simulink model "mcb_pmsm_nonlin_fwc"  (R2024b)
settings: Solver=FixedStepDiscrete  StartTime=0.0  StopTime=inf  RelTol=1e-3  EnableMultiTasking=on
InitFcn:
  | mcb_e11_nonlin_fwc_data;
model workspace (MAT data in the model file):
  encoderResolution = 2000
  hallOffset = '0.5'
  indexOffset = 850
  polePairs = '4'
values from neighbouring files (symbols this model uses):
  PI_params = mcb_SetControllerParameters(pmsm,inverter,PU_System,T_pwm,Ts,Ts_speed,Delays)    [mcb_pmsm_nonlin_fwc_data.m]
  pmsm =     [IPMSM_template_data.mat]    (also in mcb_pmsm_nonlin_fwc_data.m = mcbPMSMUpdateLdLqFluxPM(pmsm,PMSMLUT,round(tmpmat(1,1)),roun)
  PU_System = mcb_SetPUSystem(pmsm,inverter)    [mcb_pmsm_nonlin_fwc_data.m]
  PWM_frequency = 20e3    (= 20000)    [mcb_pmsm_nonlin_fwc_data.m]
  Ts = T_pwm    (= 5e-05)    [mcb_pmsm_nonlin_fwc_data.m]
  Ts_motor = T_pwm/2    (= 2.5e-05)    [mcb_pmsm_nonlin_fwc_data.m]
  Ts_speed = 30*Ts    (= 0.0015)    [mcb_pmsm_nonlin_fwc_data.m]
libraries: nesl_utility x11, mcbcontrolslib x9, fl_lib x8, ee_lib x7, slpidlib x3, mcbpmsmnonlinearlib x3, mcbpositiondecoderlib x2, nesl_utility_internal x2, simulink x1, eeGeneralControl x1, mcbutilslib x1
(part 2 of 2)

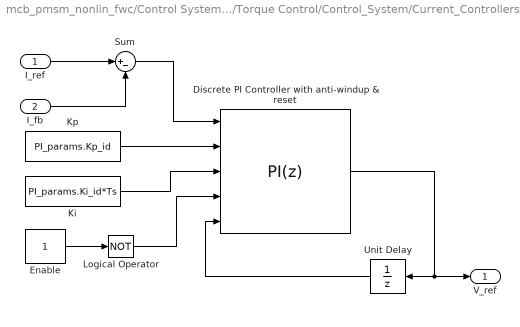
== system mcb_pmsm_nonlin_fwc/Control System/Torque Control/Control_System/Current_Controllers/PI_Controller_Id ==
  I_ref : Inport
  I_fb : Inport  Port=2
  Discrete PI Controller with anti-windup & reset : slpidlib/PID Controller  Controller=PI  Form=Parallel  TimeDomain=Discrete-time  UseExternalTs=off  SampleTime=-1  IntegratorMethod=Forward Euler  FilterMethod=Forward Euler  ControllerParametersSource=external  P=1  I=1  UseKiTs=on  D=0  UseExternalDerivativeSource=off  N=100  UseFilter=on  TunerSelectOption=Transfer Function Based (PID Tuner App)  InitialConditionSource=external  InitialConditionForIntegrator=0  InitialConditionForFilter=0  DifferentiatorICPrevScaledInput=0  ExternalReset=level  TrackingMode=off  Kt=1  LimitOutput=on  SatLimitsSource=internal  UpperSaturationLimit=1  LowerSaturationLimit=-1  LinearizeAsGain=on  AntiWindupMode=clamping  Kb=1  LimitIntegrator=off  UpperIntegratorSaturationLimit=inf  LowerIntegratorSaturationLimit=-inf  RndMeth=Simplest  POutMin=[]  POutMax=[]  IOutMin=[]  IOutMax=[]  DOutMin=[]  DOutMax=[]  NOutMin=[]  NOutMax=[]  SumOutMin=[]  SumOutMax=[]  SaturationOutDataTypeStr=Inherit: Inherit via back propagation  SaturationOutMin=[]  SaturationOutMax=[]  PParamMin=[]  PParamMax=[]  IParamMin=[]  IParamMax=[]  DParamMin=[]  DParamMax=[]  NParamMin=[]  NParamMax=[]  KbParamMin=[]  KbParamMax=[]  KtParamMin=[]  KtParamMax=[]  KbOutMin=[]  KbOutMax=[]  KtOutMin=[]  KtOutMax=[]  IntegratorOutMin=[]  IntegratorOutMax=[]  FilterOutMin=[]  FilterOutMax=[]  SumI1OutMin=[]  SumI1OutMax=[]  SumI2OutMin=[]  SumI2OutMax=[]  SumI3OutMin=[]  SumI3OutMax=[]  SumI4OutMin=[]  SumI4OutMax=[]  SumDOutMin=[]  SumDOutMax=[]  DifferentiatorOutMin=[]  DifferentiatorOutMax=[]  FilterDiffOutCoefMin=[]  FilterDiffOutCoefMax=[]  ReciprocalOutMin=[]  ReciprocalOutMax=[]  SumDenOutMin=[]  SumDenOutMax=[]  SumNumOutMin=[]  SumNumOutMax=[]  DivideOutMin=[]  DivideOutMax=[]  UdiffTsProdOutMin=[]  UdiffTsProdOutMax=[]  NTsProdOutMin=[]  NTsProdOutMax=[]  UintegralTsProdOutMin=[]  UintegralTsProdOutMax=[]  UngainTsProdOutMin=[]  UngainTsProdOutMax=[]  ClampingZeroOutDataTypeStr=Inherit: Inherit via back propagation  ClampingZeroOutMin=[]  ClampingZeroOutMax=[]  FilterDenConstantOutDataTypeStr=Inherit: Inherit via back propagation  FilterDenConstantOutMin=[]  FilterDenConstantOutMax=[]  PCopyOutDataTypeStr=Inherit: Inherit via back propagation  PCopyOutMin=[]  PCopyOutMax=[]  NCopyOutDataTypeStr=Inherit: Inherit via back propagation  NCopyOutMin=[]  NCopyOutMax=[]  IntegratorContinuousStateAttributes=''  IntegratorStateMustResolveToSignalObject=off  IntegratorRTWStateStorageClass=Auto  FilterContinuousStateAttributes=''  FilterStateMustResolveToSignalObject=off  FilterRTWStateStorageClass=Auto  ParallelPVariant=ExternalParameters  IdealPVariant=Disabled  IVariant=ExternalParameters  DVariant=Disabled  IntegratorVariant=Discrete  SatVariant=Enabled  AWVariant=DiscClampingParallel  PCopyVariant=Disabled  TRVariant=Disabled  FdbkBlocksVariant=Forward  IdealPFdbkVariant=Disabled  SatFdbkVariant=Disabled  DerivativeFilterVariant=Disabled  NVariant=Disabled  NCopyVariant=Disabled_SignalSpec  FilterICVariant=Disabled  IntegratorICVariant=ExternalICs  ExternalResetVariant=ExternalReset  TRSumVariant=Passthrough  SumFdbkVariant=Disabled  SumVariant=Sum_PI  TsampFilterVariant=InternalTs  TsampNgainVariant=Passthrough  TsampIntegralVariant=Disabled_SignalSpec  ExternalSaturationOutDataTypeStr=Inherit: Same as second input  DerivativeSourceVariant=Disabled  PreIntVariant=InternalPreInt
  Enable : Constant  OutDataTypeStr=boolean  SampleTime=-1
  Ki : Constant  Value=PI_params.Ki_id*Ts  OutDataTypeStr=dataType  SampleTime=-1
  Kp : Constant  Value=PI_params.Kp_id  OutDataTypeStr=dataType  SampleTime=-1
  Logical Operator : Logic  Operator=NOT  IconShape=distinctive  AllPortsSameDT=off  OutDataTypeStr=boolean
  Sum : Sum  Inputs=|+-  OutDataTypeStr=Inherit: Same as first input
  Unit Delay : UnitDelay  SampleTime=-1  HasFrameUpgradeWarning=on
  V_ref : Outport  VectorParamsAs1DForOutWhenUnconnected=off
  wires:
  I_fb/1 -> Sum/2
  I_ref/1 -> Sum/1
  Ki/1 -> Discrete PI Controller with anti-windup & reset/3
  Unit Delay/1 -> Discrete PI Controller with anti-windup & reset/5
  Logical Operator/1 -> Discrete PI Controller with anti-windup & reset/4
  Sum/1 -> Discrete PI Controller with anti-windup & reset/1
  Kp/1 -> Discrete PI Controller with anti-windup & reset/2
  Discrete PI Controller with anti-windup & reset/1 -> V_ref/1, Unit Delay/1
  Enable/1 -> Logical Operator/1

== system mcb_pmsm_nonlin_fwc/Control System/Torque Control/Control_System/Current_Controllers/PI_Controller_Iq ==
  I_ref : Inport
  I_fb : Inport  Port=2
  Discrete PI Controller with anti-windup & reset : slpidlib/PID Controller  Controller=PI  Form=Parallel  TimeDomain=Discrete-time  UseExternalTs=off  SampleTime=-1  IntegratorMethod=Forward Euler  FilterMethod=Forward Euler  ControllerParametersSource=external  P=1  I=1  UseKiTs=on  D=0  UseExternalDerivativeSource=off  N=100  UseFilter=on  TunerSelectOption=Transfer Function Based (PID Tuner App)  InitialConditionSource=external  InitialConditionForIntegrator=0  InitialConditionForFilter=0  DifferentiatorICPrevScaledInput=0  ExternalReset=level  TrackingMode=off  Kt=1  LimitOutput=on  SatLimitsSource=internal  UpperSaturationLimit=1  LowerSaturationLimit=-1  LinearizeAsGain=on  AntiWindupMode=clamping  Kb=1  LimitIntegrator=off  UpperIntegratorSaturationLimit=inf  LowerIntegratorSaturationLimit=-inf  RndMeth=Simplest  POutMin=[]  POutMax=[]  IOutMin=[]  IOutMax=[]  DOutMin=[]  DOutMax=[]  NOutMin=[]  NOutMax=[]  SumOutMin=[]  SumOutMax=[]  SaturationOutDataTypeStr=Inherit: Inherit via back propagation  SaturationOutMin=[]  SaturationOutMax=[]  PParamMin=[]  PParamMax=[]  IParamMin=[]  IParamMax=[]  DParamMin=[]  DParamMax=[]  NParamMin=[]  NParamMax=[]  KbParamMin=[]  KbParamMax=[]  KtParamMin=[]  KtParamMax=[]  KbOutMin=[]  KbOutMax=[]  KtOutMin=[]  KtOutMax=[]  IntegratorOutMin=[]  IntegratorOutMax=[]  FilterOutMin=[]  FilterOutMax=[]  SumI1OutMin=[]  SumI1OutMax=[]  SumI2OutMin=[]  SumI2OutMax=[]  SumI3OutMin=[]  SumI3OutMax=[]  SumI4OutMin=[]  SumI4OutMax=[]  SumDOutMin=[]  SumDOutMax=[]  DifferentiatorOutMin=[]  DifferentiatorOutMax=[]  FilterDiffOutCoefMin=[]  FilterDiffOutCoefMax=[]  ReciprocalOutMin=[]  ReciprocalOutMax=[]  SumDenOutMin=[]  SumDenOutMax=[]  SumNumOutMin=[]  SumNumOutMax=[]  DivideOutMin=[]  DivideOutMax=[]  UdiffTsProdOutMin=[]  UdiffTsProdOutMax=[]  NTsProdOutMin=[]  NTsProdOutMax=[]  UintegralTsProdOutMin=[]  UintegralTsProdOutMax=[]  UngainTsProdOutMin=[]  UngainTsProdOutMax=[]  ClampingZeroOutDataTypeStr=Inherit: Inherit via back propagation  ClampingZeroOutMin=[]  ClampingZeroOutMax=[]  FilterDenConstantOutDataTypeStr=Inherit: Inherit via back propagation  FilterDenConstantOutMin=[]  FilterDenConstantOutMax=[]  PCopyOutDataTypeStr=Inherit: Inherit via back propagation  PCopyOutMin=[]  PCopyOutMax=[]  NCopyOutDataTypeStr=Inherit: Inherit via back propagation  NCopyOutMin=[]  NCopyOutMax=[]  IntegratorContinuousStateAttributes=''  IntegratorStateMustResolveToSignalObject=off  IntegratorRTWStateStorageClass=Auto  FilterContinuousStateAttributes=''  FilterStateMustResolveToSignalObject=off  FilterRTWStateStorageClass=Auto  ParallelPVariant=ExternalParameters  IdealPVariant=Disabled  IVariant=ExternalParameters  DVariant=Disabled  IntegratorVariant=Discrete  SatVariant=Enabled  AWVariant=DiscClampingParallel  PCopyVariant=Disabled  TRVariant=Disabled  FdbkBlocksVariant=Forward  IdealPFdbkVariant=Disabled  SatFdbkVariant=Disabled  DerivativeFilterVariant=Disabled  NVariant=Disabled  NCopyVariant=Disabled_SignalSpec  FilterICVariant=Disabled  IntegratorICVariant=ExternalICs  ExternalResetVariant=ExternalReset  TRSumVariant=Passthrough  SumFdbkVariant=Disabled  SumVariant=Sum_PI  TsampFilterVariant=InternalTs  TsampNgainVariant=Passthrough  TsampIntegralVariant=Disabled_SignalSpec  ExternalSaturationOutDataTypeStr=Inherit: Same as second input  DerivativeSourceVariant=Disabled  PreIntVariant=InternalPreInt
  Enable : Constant  OutDataTypeStr=boolean  SampleTime=-1
  Ki : Constant  Value=PI_params.Ki_i*Ts  OutDataTypeStr=dataType  SampleTime=-1
  Kp : Constant  Value=PI_params.Kp_i  OutDataTypeStr=dataType  SampleTime=-1
  Logical Operator : Logic  Operator=NOT  IconShape=distinctive  AllPortsSameDT=off  OutDataTypeStr=boolean
  Sum : Sum  Inputs=|+-  OutDataTypeStr=Inherit: Same as first input
  Unit Delay : UnitDelay  SampleTime=-1  HasFrameUpgradeWarning=on
  V_ref : Outport  VectorParamsAs1DForOutWhenUnconnected=off
  wires:
  I_fb/1 -> Sum/2
  I_ref/1 -> Sum/1
  Ki/1 -> Discrete PI Controller with anti-windup & reset/3
  Unit Delay/1 -> Discrete PI Controller with anti-windup & reset/5
  Logical Operator/1 -> Discrete PI Controller with anti-windup & reset/4
  Sum/1 -> Discrete PI Controller with anti-windup & reset/1
  Kp/1 -> Discrete PI Controller with anti-windup & reset/2
  Discrete PI Controller with anti-windup & reset/1 -> V_ref/1, Unit Delay/1
  Enable/1 -> Logical Operator/1
